simulink model "ieee13_digital_twin"  (R2025a)
settings: Solver=FixedStepDiscrete  StartTime=0.0  StopTime=10.0  FixedStep=50e-6  RelTol=1e-3
undefined symbols (not defined in the file or in its folder): D1, Delta
libraries: spsGroundLib x21, spsSeriesRLCLoadLib x18, spsThreePhasePISectionLineLib x10, spsSeriesRLCBranchLib x8, spsThreePhaseBreakerLib x3, spsThreePhaseVIMeasurementLib x3, spsThreePhaseSourceLib x1, spsThreePhaseTransformerTwoWindingsLib x1, spspowerguiLib x1
settings Model: Creator=hari2  LastModifiedBy=munib

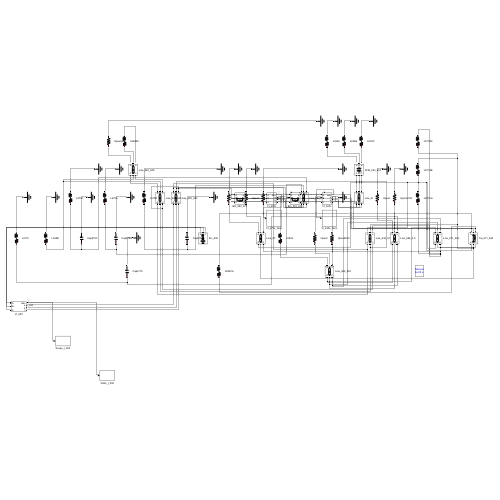
[thumbnail: Simulink's stored preview of the top-level diagram]
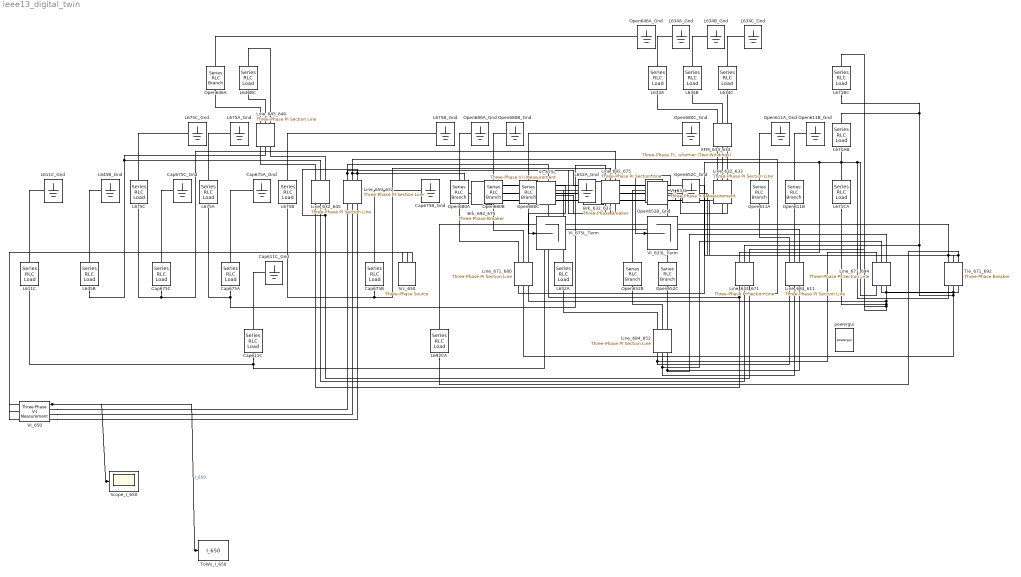
== system ieee13_digital_twin ==
  Brk_632_633 : spsThreePhaseBreakerLib/Three-Phase Breaker  InitialState=closed  SwitchA=on  SwitchB=on  SwitchC=on  SwitchTimes=[1e6]  External=off  BreakerResistance=0.01  SnubberResistance=1e6  SnubberCapacitance=inf  Measurements=None
  Brk_692_675 : spsThreePhaseBreakerLib/Three-Phase Breaker  InitialState=closed  SwitchA=on  SwitchB=on  SwitchC=on  SwitchTimes=[1e6]  External=off  BreakerResistance=0.01  SnubberResistance=1e6  SnubberCapacitance=inf  Measurements=None
  Cap611C : spsSeriesRLCLoadLib/Series RLC Load  LConnTagsString=a  RConnTagsString=__new0  NominalVoltage=2400  NominalFrequency=60  ActivePower=0  InductivePower=0  CapacitivePower=100000  Setx0=off  InitialVoltage=0  SetiL0=off  InitialCurrent=0  Measurements=None  LoadType=constant Z
  Cap611C_Gnd : spsGroundLib/Ground  LConnTagsString=a
  Cap675A : spsSeriesRLCLoadLib/Series RLC Load  LConnTagsString=a  RConnTagsString=__new0  NominalVoltage=2400  NominalFrequency=60  ActivePower=0  InductivePower=0  CapacitivePower=200000  Setx0=off  InitialVoltage=0  SetiL0=off  InitialCurrent=0  Measurements=None  LoadType=constant Z
  Cap675A_Gnd : spsGroundLib/Ground  LConnTagsString=a
  Cap675B : spsSeriesRLCLoadLib/Series RLC Load  LConnTagsString=a  RConnTagsString=__new0  NominalVoltage=2400  NominalFrequency=60  ActivePower=0  InductivePower=0  CapacitivePower=200000  Setx0=off  InitialVoltage=0  SetiL0=off  InitialCurrent=0  Measurements=None  LoadType=constant Z
  Cap675B_Gnd : spsGroundLib/Ground  LConnTagsString=a
  Cap675C : spsSeriesRLCLoadLib/Series RLC Load  LConnTagsString=a  RConnTagsString=__new0  NominalVoltage=2400  NominalFrequency=60  ActivePower=0  InductivePower=0  CapacitivePower=200000  Setx0=off  InitialVoltage=0  SetiL0=off  InitialCurrent=0  Measurements=None  LoadType=constant Z
  Cap675C_Gnd : spsGroundLib/Ground  LConnTagsString=a
  L611C : spsSeriesRLCLoadLib/Series RLC Load  LConnTagsString=a  RConnTagsString=__new0  NominalVoltage=2400  NominalFrequency=60  ActivePower=170000  InductivePower=80000  CapacitivePower=0  Setx0=off  InitialVoltage=0  SetiL0=off  InitialCurrent=0  Measurements=None  LoadType=constant I
  L611C_Gnd : spsGroundLib/Ground  LConnTagsString=a
  L634A : spsSeriesRLCLoadLib/Series RLC Load  LConnTagsString=a  RConnTagsString=__new0  NominalVoltage=480/sqrt(3)  NominalFrequency=60  ActivePower=160000  InductivePower=110000  CapacitivePower=0  Setx0=off  InitialVoltage=0  SetiL0=off  InitialCurrent=0  Measurements=None  LoadType=constant PQ
  L634A_Gnd : spsGroundLib/Ground  LConnTagsString=a
  L634B : spsSeriesRLCLoadLib/Series RLC Load  LConnTagsString=a  RConnTagsString=__new0  NominalVoltage=480/sqrt(3)  NominalFrequency=60  ActivePower=120000  InductivePower=90000  CapacitivePower=0  Setx0=off  InitialVoltage=0  SetiL0=off  InitialCurrent=0  Measurements=None  LoadType=constant PQ
  L634B_Gnd : spsGroundLib/Ground  LConnTagsString=a
  L634C : spsSeriesRLCLoadLib/Series RLC Load  LConnTagsString=a  RConnTagsString=__new0  NominalVoltage=480/sqrt(3)  NominalFrequency=60  ActivePower=120000  InductivePower=90000  CapacitivePower=0  Setx0=off  InitialVoltage=0  SetiL0=off  InitialCurrent=0  Measurements=None  LoadType=constant PQ
  L634C_Gnd : spsGroundLib/Ground  LConnTagsString=a
  L645B : spsSeriesRLCLoadLib/Series RLC Load  LConnTagsString=a  RConnTagsString=__new0  NominalVoltage=2400  NominalFrequency=60  ActivePower=170000  InductivePower=125000  CapacitivePower=0  Setx0=off  InitialVoltage=0  SetiL0=off  InitialCurrent=0  Measurements=None  LoadType=constant PQ
  L645B_Gnd : spsGroundLib/Ground  LConnTagsString=a
  L646BC : spsSeriesRLCLoadLib/Series RLC Load  LConnTagsString=a  RConnTagsString=__new0  NominalVoltage=4160  NominalFrequency=60  ActivePower=230000  InductivePower=132000  CapacitivePower=0  Setx0=off  InitialVoltage=0  SetiL0=off  InitialCurrent=0  Measurements=None  LoadType=constant Z
  L652A : spsSeriesRLCLoadLib/Series RLC Load  LConnTagsString=a  RConnTagsString=__new0  NominalVoltage=2400  NominalFrequency=60  ActivePower=128000  InductivePower=86000  CapacitivePower=0  Setx0=off  InitialVoltage=0  SetiL0=off  InitialCurrent=0  Measurements=None  LoadType=constant Z
  L652A_Gnd : spsGroundLib/Ground  LConnTagsString=a
  L671AB : spsSeriesRLCLoadLib/Series RLC Load  LConnTagsString=a  RConnTagsString=__new0  NominalVoltage=4160  NominalFrequency=60  ActivePower=385000  InductivePower=220000  CapacitivePower=0  Setx0=off  InitialVoltage=0  SetiL0=off  InitialCurrent=0  Measurements=None  LoadType=constant PQ
  L671BC : spsSeriesRLCLoadLib/Series RLC Load  LConnTagsString=a  RConnTagsString=__new0  NominalVoltage=4160  NominalFrequency=60  ActivePower=385000  InductivePower=220000  CapacitivePower=0  Setx0=off  InitialVoltage=0  SetiL0=off  InitialCurrent=0  Measurements=None  LoadType=constant PQ
  L671CA : spsSeriesRLCLoadLib/Series RLC Load  LConnTagsString=a  RConnTagsString=__new0  NominalVoltage=4160  NominalFrequency=60  ActivePower=385000  InductivePower=220000  CapacitivePower=0  Setx0=off  InitialVoltage=0  SetiL0=off  InitialCurrent=0  Measurements=None  LoadType=constant PQ
  L675A : spsSeriesRLCLoadLib/Series RLC Load  LConnTagsString=a  RConnTagsString=__new0  NominalVoltage=2400  NominalFrequency=60  ActivePower=485000  InductivePower=190000  CapacitivePower=0  Setx0=off  InitialVoltage=0  SetiL0=off  InitialCurrent=0  Measurements=None  LoadType=constant PQ
  L675A_Gnd : spsGroundLib/Ground  LConnTagsString=a
  L675B : spsSeriesRLCLoadLib/Series RLC Load  LConnTagsString=a  RConnTagsString=__new0  NominalVoltage=2400  NominalFrequency=60  ActivePower=68000  InductivePower=60000  CapacitivePower=0  Setx0=off  InitialVoltage=0  SetiL0=off  InitialCurrent=0  Measurements=None  LoadType=constant PQ
  L675B_Gnd : spsGroundLib/Ground  LConnTagsString=a
  L675C : spsSeriesRLCLoadLib/Series RLC Load  LConnTagsString=a  RConnTagsString=__new0  NominalVoltage=2400  NominalFrequency=60  ActivePower=290000  InductivePower=212000  CapacitivePower=0  Setx0=off  InitialVoltage=0  SetiL0=off  InitialCurrent=0  Measurements=None  LoadType=constant PQ
  L675C_Gnd : spsGroundLib/Ground  LConnTagsString=a
  L692CA : spsSeriesRLCLoadLib/Series RLC Load  LConnTagsString=a  RConnTagsString=__new0  NominalVoltage=4160  NominalFrequency=60  ActivePower=170000  InductivePower=151000  CapacitivePower=0  Setx0=off  InitialVoltage=0  SetiL0=off  InitialCurrent=0  Measurements=None  LoadType=constant I
  Line_632_633 : spsThreePhasePISectionLineLib/Three-Phase PI Section Line  LConnTagsString=a|b|c  RConnTagsString=A|B|C  Length=0.152400  Frequency=60  Resistances=[0.467643959277818 1.16910989819454]  Inductances=[0.00194722870280028 0.00486807175700071]  Capacitances=[9.39330995197123e-09 4.69665497598562e-09]
  Line_632_645 : spsThreePhasePISectionLineLib/Three-Phase PI Section Line  LConnTagsString=a|b|c  RConnTagsString=A|B|C  Length=0.152400  Frequency=60  Resistances=[0.826050862960312 2.06512715740078]  Inductances=[0.00222034178562914 0.00555085446407284]  Capacitances=[7.76270782256517e-09 3.88135391128259e-09]
  Line_632_671 : spsThreePhasePISectionLineLib/Three-Phase PI Section Line  LConnTagsString=a|b|c  RConnTagsString=A|B|C  Length=0.609600  Frequency=60  Resistances=[0.215305118110236 0.538262795275591]  Inductances=[0.00167774174418521 0.00419435436046303]  Capacitances=[1.03835715099892e-08 5.19178575499459e-09]
  Line_645_646 : spsThreePhasePISectionLineLib/Three-Phase PI Section Line  LConnTagsString=a|b|c  RConnTagsString=A|B|C  Length=0.091440  Frequency=60  Resistances=[0.826050862960312 2.06512715740078]  Inductances=[0.00222034178562914 0.00555085446407284]  Capacitances=[7.76270782256517e-09 3.88135391128259e-09]
  Line_650_632 : spsThreePhasePISectionLineLib/Three-Phase PI Section Line  LConnTagsString=a|b|c  RConnTagsString=A|B|C  Length=0.609600  Frequency=60  Resistances=[0.215305118110236 0.538262795275591]  Inductances=[0.00167774174418521 0.00419435436046303]  Capacitances=[1.03835715099892e-08 5.19178575499459e-09]
  Line_671_680 : spsThreePhasePISectionLineLib/Three-Phase PI Section Line  LConnTagsString=a|b|c  RConnTagsString=A|B|C  Length=0.304800  Frequency=60  Resistances=[0.215305118110236 0.538262795275591]  Inductances=[0.00167774174418521 0.00419435436046303]  Capacitances=[1.03835715099892e-08 5.19178575499459e-09]
  Line_671_684 : spsThreePhasePISectionLineLib/Three-Phase PI Section Line  LConnTagsString=a|b|c  RConnTagsString=A|B|C  Length=0.091440  Frequency=60  Resistances=[0.821949813091545 2.05487453272886]  Inductances=[0.00223649452076325 0.00559123630190813]  Capacitances=[7.58189608335983e-09 3.79094804167991e-09]
  Line_684_611 : spsThreePhasePISectionLineLib/Three-Phase PI Section Line  LConnTagsString=a|b|c  RConnTagsString=A|B|C  Length=0.091440  Frequency=60  Resistances=[0.825926588721864 2.06481647180466]  Inductances=[0.00222100108094073 0.00555250270235183]  Capacitances=[7.74671991125896e-09 3.87335995562948e-09]
  Line_684_652 : spsThreePhasePISectionLineLib/Three-Phase PI Section Line  LConnTagsString=a|b|c  RConnTagsString=A|B|C  Length=0.243840  Frequency=60  Resistances=[0.834190825578621 2.08547706394655]  Inductances=[0.000849502008992099 0.00212375502248025]  Capacitances=[1.45044968551232e-07 7.25224842756158e-08]
  Line_692_675 : spsThreePhasePISectionLineLib/Three-Phase PI Section Line  LConnTagsString=a|b|c  RConnTagsString=A|B|C  Length=0.152400  Frequency=60  Resistances=[0.49597848564384 1.2399462141096]  Inductances=[0.000735608743913803 0.00183902185978451]  Capacitances=[1.58230874783162e-07 7.91154373915808e-08]
  Open611A : spsSeriesRLCBranchLib/Series RLC Branch  LConnTagsString=__new0  RConnTagsString=__new0  BranchType=R  Resistance=1e6  Inductance=1e-3  SetiL0=off  InitialCurrent=0  Capacitance=1e-6  Setx0=off  InitialVoltage=0  Measurements=None
  Open611A_Gnd : spsGroundLib/Ground  LConnTagsString=a
  Open611B : spsSeriesRLCBranchLib/Series RLC Branch  LConnTagsString=__new0  RConnTagsString=__new0  BranchType=R  Resistance=1e6  Inductance=1e-3  SetiL0=off  InitialCurrent=0  Capacitance=1e-6  Setx0=off  InitialVoltage=0  Measurements=None
  Open611B_Gnd : spsGroundLib/Ground  LConnTagsString=a
  Open646A : spsSeriesRLCBranchLib/Series RLC Branch  LConnTagsString=__new0  RConnTagsString=__new0  BranchType=R  Resistance=1e6  Inductance=1e-3  SetiL0=off  InitialCurrent=0  Capacitance=1e-6  Setx0=off  InitialVoltage=0  Measurements=None
  Open646A_Gnd : spsGroundLib/Ground  LConnTagsString=a
  Open652B : spsSeriesRLCBranchLib/Series RLC Branch  LConnTagsString=__new0  RConnTagsString=__new0  BranchType=R  Resistance=1e6  Inductance=1e-3  SetiL0=off  InitialCurrent=0  Capacitance=1e-6  Setx0=off  InitialVoltage=0  Measurements=None
  Open652B_Gnd : spsGroundLib/Ground  LConnTagsString=a
  Open652C : spsSeriesRLCBranchLib/Series RLC Branch  LConnTagsString=__new0  RConnTagsString=__new0  BranchType=R  Resistance=1e6  Inductance=1e-3  SetiL0=off  InitialCurrent=0  Capacitance=1e-6  Setx0=off  InitialVoltage=0  Measurements=None
  Open652C_Gnd : spsGroundLib/Ground  LConnTagsString=a
  Open680A : spsSeriesRLCBranchLib/Series RLC Branch  LConnTagsString=__new0  RConnTagsString=__new0  BranchType=R  Resistance=1e6  Inductance=1e-3  SetiL0=off  InitialCurrent=0  Capacitance=1e-6  Setx0=off  InitialVoltage=0  Measurements=None
  Open680A_Gnd : spsGroundLib/Ground  LConnTagsString=a
  Open680B : spsSeriesRLCBranchLib/Series RLC Branch  LConnTagsString=__new0  RConnTagsString=__new0  BranchType=R  Resistance=1e6  Inductance=1e-3  SetiL0=off  InitialCurrent=0  Capacitance=1e-6  Setx0=off  InitialVoltage=0  Measurements=None
  Open680B_Gnd : spsGroundLib/Ground  LConnTagsString=a
  Open680C : spsSeriesRLCBranchLib/Series RLC Branch  LConnTagsString=__new0  RConnTagsString=__new0  BranchType=R  Resistance=1e6  Inductance=1e-3  SetiL0=off  InitialCurrent=0  Capacitance=1e-6  Setx0=off  InitialVoltage=0  Measurements=None
  Open680C_Gnd : spsGroundLib/Ground  LConnTagsString=a
  Scope_I_650 : Scope
  Src_650 : spsThreePhaseSourceLib/Three-Phase Source  InternalConnection=Yg  VoltagePhases=off  Voltage=4160  PhaseAngle=0  Voltage_phases=[25e3 25e3 25e3]/sqrt(3)  PhaseAngles_phases=[0 -120 +120]  Frequency=60  NonIdealSource=on  SpecifyImpedance=off  Resistance=0.1  Inductance=0.001  ShortCircuitLevel=100e6  BaseVoltage=25e3  XRratio=7  BusType=swing  Pref=10e3  Qref=0  Prefabc=[10e3, 10e3, 10e3]  Qrefabc=[0, 0, 0]  Qmin=-inf  Qmax=inf
  Tie_671_692 : spsThreePhaseBreakerLib/Three-Phase Breaker  InitialState=closed  SwitchA=on  SwitchB=on  SwitchC=on  SwitchTimes=[1e6]  External=off  BreakerResistance=0.01  SnubberResistance=1e6  SnubberCapacitance=inf  Measurements=None
  ToWs_I_650 : ToWorkspace  VariableName=I_650  SaveFormat=Timeseries  SampleTime=-1
  VI_633L : spsThreePhaseVIMeasurementLib/Three-Phase V-I Measurement  VoltageMeasurement=no  SetLabelV=off  LabelV=Vabc  Vpu=off  VpuLL=off  CurrentMeasurement=yes  SetLabelI=off  LabelI=Iabc  Ipu=off  Pbase=100e6  Vbase=500e3  OutputType=Complex  PhasorSimulation=off  PSBequivalent=0
  VI_633L_Term : Terminator
  VI_650 : spsThreePhaseVIMeasurementLib/Three-Phase V-I Measurement  VoltageMeasurement=no  SetLabelV=off  LabelV=Vabc  Vpu=off  VpuLL=off  CurrentMeasurement=yes  SetLabelI=off  LabelI=Iabc  Ipu=off  Pbase=100e6  Vbase=500e3  OutputType=Complex  PhasorSimulation=off  PSBequivalent=0
  VI_675L : spsThreePhaseVIMeasurementLib/Three-Phase V-I Measurement  VoltageMeasurement=no  SetLabelV=off  LabelV=Vabc  Vpu=off  VpuLL=off  CurrentMeasurement=yes  SetLabelI=off  LabelI=Iabc  Ipu=off  Pbase=100e6  Vbase=500e3  OutputType=Complex  PhasorSimulation=off  PSBequivalent=0
  VI_675L_Term : Terminator
  XFM_633_634 : spsThreePhaseTransformerTwoWindingsLib/Three-Phase Transformer (Two Windings)  Winding1Connection=Delta (D1)  Winding2Connection=Yg  CoreType=Three single-phase transformers  SetSaturation=off  Hysteresis=off  DataFile='hysteresis'  SetInitialFlux=off  Measurements=None  UNITS=pu  NominalPower=[500000 60]  Winding1=[4160 0.0055 0.01]  Winding2=[480 0.0055 0.01]  Rm=500  Lm=500  L0=0.5  Saturation=[ 0,0 ; 0.0024,1.2 ; 1.0,1.52 ]  InitialFluxes=[ 0.8 , -0.8 , 0.7 ]  BreakLoop=off  DiscreteSolver=Trapezoidal iterative  DataType=off  TransfoNumber=1
  powergui : spspowerguiLib/powergui  Priority=1  SimulationMode=Discrete  SampleTime=50e-6  frequency=60  Iterations=50  frequencyindice=60  Pbase=100e6  ErrMax=1e-4  UnitsV=kV  UnitsW=MW  buscounter=0  FunctionMessages=off  echomessages=off  EnableUseOfTLC=off  CurrentSourceSwitches=off  DisableSnubberDevices=off  DisableRonSwitches=off  DisableVfSwitches=off  DisplayEquations=off  AutomaticDiscreteSolvers=off  SolverType=Tustin/Backward Euler (TBE)  Interpol=off  ExternalGateDelay=off  methode=off  Ts=100  x0status=blocks  SPID=on  SwTol=0  HookPort=off  NonlinearTolerance=1e-4  nMaxIteration=100  ContinueOnMaxIteration=off  RestoreLinks=warning  ResistiveCurrentMeasurement=off  Frange=[0:2:500]  Ylog=off  Xlog=on  ShowGrid=off  save=off  variable=ZData  structure=0  ZoomFFT=off  StartTime=0.0  cycles=1  DisplayStyle=1  fundamental=60  FreqAxis=off  MaxFrequency=1000  frequencyindicesteady=1  RmsSteady=1  display=off
  wires:
  VI_650/1 -> Scope_I_650/1, ToWs_I_650/1  "I_650"
  VI_633L/1 -> VI_633L_Term/1
  VI_675L/1 -> VI_675L_Term/1
  connections:
  Open680B/RConn1 -- Open680B_Gnd/LConn1
  Line_684_652/RConn1 -- L652A/LConn1
  L652A/RConn1 -- L652A_Gnd/LConn1
  Cap611C/LConn1 -- L611C/LConn1 -- Line_684_611/RConn3
  Line_684_652/LConn2 -- Line_671_684/RConn2 -- Line_684_611/LConn2
  Line_645_646/RConn3 -- L646BC/RConn1
  Line_684_652/LConn1 -- Line_684_611/LConn1 -- Line_671_684/RConn1
  Line_684_652/LConn3 -- Line_684_611/LConn3 -- Line_671_684/RConn3
  XFM_633_634/RConn2 -- L634B/LConn1
  Open680A/RConn1 -- Open680A_Gnd/LConn1
  Cap611C/RConn1 -- Cap611C_Gnd/LConn1
  Line_684_652/RConn2 -- Open652B/LConn1
  Line_684_652/RConn3 -- Open652C/LConn1
  L645B/LConn1 -- Line_645_646/LConn2 -- Line_632_645/RConn2
  Line_645_646/RConn1 -- Open646A/LConn1
  Cap675B/LConn1 -- L675B/LConn1 -- Line_692_675/RConn2
  Cap675C/LConn1 -- L675C/LConn1 -- Line_692_675/RConn3
  L675C/RConn1 -- L675C_Gnd/LConn1
  Cap675A/LConn1 -- L675A/LConn1 -- Line_692_675/RConn1
  Line_632_671/LConn3 -- Line_632_645/LConn3 -- Line_650_632/RConn3 -- Brk_632_633/LConn3
  L675A/RConn1 -- L675A_Gnd/LConn1
  Line_632_671/LConn2 -- Line_632_645/LConn2 -- Line_650_632/RConn2 -- Brk_632_633/LConn2
  Open652B/RConn1 -- Open652B_Gnd/LConn1
  Line_671_680/RConn3 -- Open680C/LConn1
  L611C/RConn1 -- L611C_Gnd/LConn1
  L645B/RConn1 -- L645B_Gnd/LConn1
  Cap675B/RConn1 -- Cap675B_Gnd/LConn1
  Cap675C/RConn1 -- Cap675C_Gnd/LConn1
  Cap675A/RConn1 -- Cap675A_Gnd/LConn1
  Line_645_646/RConn2 -- L646BC/LConn1
  Line_671_680/RConn1 -- Open680A/LConn1
  Line_671_680/RConn2 -- Open680B/LConn1
  Open652C/RConn1 -- Open652C_Gnd/LConn1
  Line_684_611/RConn1 -- Open611A/LConn1
  Line_684_611/RConn2 -- Open611B/LConn1
  L671CA/RConn1 -- Line_671_684/LConn1 -- Tie_671_692/LConn1 -- Line_671_680/LConn1 -- Line_632_671/RConn1 -- L671AB/LConn1
  L671CA/LConn1 -- L671BC/RConn1 -- Line_632_671/RConn3 -- Tie_671_692/LConn3 -- Line_671_684/LConn3 -- Line_671_680/LConn3
  L675B/RConn1 -- L675B_Gnd/LConn1
  L634A/RConn1 -- L634A_Gnd/LConn1
  Open646A/RConn1 -- Open646A_Gnd/LConn1
  Line_632_645/RConn1 -- Line_645_646/LConn1
  Line_632_645/RConn3 -- Line_645_646/LConn3
  Open680C/RConn1 -- Open680C_Gnd/LConn1
  Line_632_633/RConn1 -- XFM_633_634/LConn1
  Line_632_633/RConn2 -- XFM_633_634/LConn2
  Line_632_633/RConn3 -- XFM_633_634/LConn3
  Open611A/RConn1 -- Open611A_Gnd/LConn1
  Open611B/RConn1 -- Open611B_Gnd/LConn1
  XFM_633_634/RConn1 -- L634A/LConn1
  XFM_633_634/RConn3 -- L634C/LConn1
  L671BC/LConn1 -- Line_671_684/LConn2 -- Tie_671_692/LConn2 -- Line_671_680/LConn2 -- Line_632_671/RConn2 -- L671AB/RConn1
  L634B/RConn1 -- L634B_Gnd/LConn1
  L634C/RConn1 -- L634C_Gnd/LConn1
  Src_650/RConn1 -- VI_650/LConn1
  VI_650/RConn1 -- Line_650_632/LConn1
  Src_650/RConn2 -- VI_650/LConn2
  VI_650/RConn2 -- Line_650_632/LConn2
  Src_650/RConn3 -- VI_650/LConn3
  VI_650/RConn3 -- Line_650_632/LConn3
  Line_632_645/LConn1 -- Line_632_671/LConn1 -- Line_650_632/RConn1 -- Brk_632_633/LConn1
  Brk_632_633/RConn1 -- VI_633L/LConn1
  VI_633L/RConn1 -- Line_632_633/LConn1
  Brk_632_633/RConn2 -- VI_633L/LConn2
  VI_633L/RConn2 -- Line_632_633/LConn2
  Brk_632_633/RConn3 -- VI_633L/LConn3
  VI_633L/RConn3 -- Line_632_633/LConn3
  Tie_671_692/RConn1 -- L692CA/RConn1 -- Brk_692_675/LConn1
  Tie_671_692/RConn3 -- L692CA/LConn1 -- Brk_692_675/LConn3
  Brk_692_675/RConn1 -- VI_675L/LConn1
  VI_675L/RConn1 -- Line_692_675/LConn1
  Tie_671_692/RConn2 -- Brk_692_675/LConn2
  Brk_692_675/RConn2 -- VI_675L/LConn2
  VI_675L/RConn2 -- Line_692_675/LConn2
  Brk_692_675/RConn3 -- VI_675L/LConn3
  VI_675L/RConn3 -- Line_692_675/LConn3
